simulink model "finalmodel3"  (R2024b)
settings: Solver=ode4  StartTime=0.0  StopTime=110.0  FixedStep=SampleTime  MaxStep=1e-3  RelTol=1e-4  AbsTol=1e-3
PreLoadFcn:
  | load('finalmodel3.mat');
InitFcn:
  | if exist('finalmodel3.mat','file'), load('finalmodel3.mat'); end
values from neighbouring files (symbols this model uses):
  den_d = [1 -0.993736492083]    [finalmodel2.mat]    (also in finalmodel3.mat)
  Dp = 6191.85011148    [finalmodel2.mat]    (also in finalmodel3.mat)
  Dq = 673609.679265    [finalmodel2.mat]    (also in finalmodel3.mat)
  fg = 60    [finalmodel2.mat]    (also in finalmodel3.mat)
  k10 = 1    [finalmodel2.mat]    (also in finalmodel3.mat)
  k11 = 25    [finalmodel2.mat]    (also in finalmodel3.mat)
  k12 = 1    [finalmodel2.mat]    (also in finalmodel3.mat)
  k13 = 120    [finalmodel2.mat]    (also in finalmodel3.mat)
  k14 = 1    [finalmodel2.mat]    (also in finalmodel3.mat)
  k2 = 9.4    [finalmodel2.mat]    (also in finalmodel3.mat)
  k3 = 1    [finalmodel2.mat]    (also in finalmodel3.mat)
  k4 = 25    [finalmodel2.mat]    (also in finalmodel3.mat)
  k5 = 1    [finalmodel2.mat]    (also in finalmodel3.mat)
  k6 = 120    [finalmodel2.mat]    (also in finalmodel3.mat)
  k7 = 1    [finalmodel2.mat]    (also in finalmodel3.mat)
  k9 = 9.4    [finalmodel2.mat]    (also in finalmodel3.mat)
  Ki = 9    [finalmodel2.mat]    (also in finalmodel3.mat)
  Kp = 1    [finalmodel2.mat]    (also in finalmodel3.mat)
  L = 5.78745247607e-06    [finalmodel2.mat]    (also in finalmodel3.mat)
  num_d = [0.00313175395836 0.00313175395836]    [finalmodel2.mat]    (also in finalmodel3.mat)
  Pset = 8281000    [finalmodel2.mat]    (also in finalmodel3.mat = 8280000)
  Qset = 0    [finalmodel2.mat]    (also in finalmodel3.mat)
  R = 0.000290909090909    [finalmodel2.mat]    (also in finalmodel3.mat)
  SampleTime = 5e-05    [finalmodel2.mat]    (also in finalmodel3.mat)
  Ts = 5e-05    [finalmodel2.mat]    (also in finalmodel3.mat)
  tv = 0.05    [finalmodel2.mat]    (also in finalmodel3.mat)
  Vdclink = 800    [finalmodel2.mat]    (also in finalmodel3.mat)
  Vnpeak = 326.598632371    [finalmodel2.mat]    (also in finalmodel3.mat)
  Wn = 376.991118431    [finalmodel2.mat]    (also in finalmodel3.mat)
undefined symbols (not defined in the file or in its folder): dspblkCoreblockFVToolHelper, gcbh, sigbuilder_block
libraries: spsThreePhaseVIMeasurementLib x15, spsLoadFlowBusLib x9, spsThreePhasePISectionLineLib x6, simulink_extras x5, spsThreePhaseTransformerTwoWindingsLib x4, spsThreePhaseParallelRLCLoadLib x4, spsThreePhaseSeriesRLCBranchLib x3, spsSynchronousMachinepuStandardLib x2, spsExcitationSystemLib x2, spsMultiBandPowerSystemStabilizerLib x2, spsSteamTurbineandGovernorLib x2, spsGroundLib x2
(part 2 of 3)

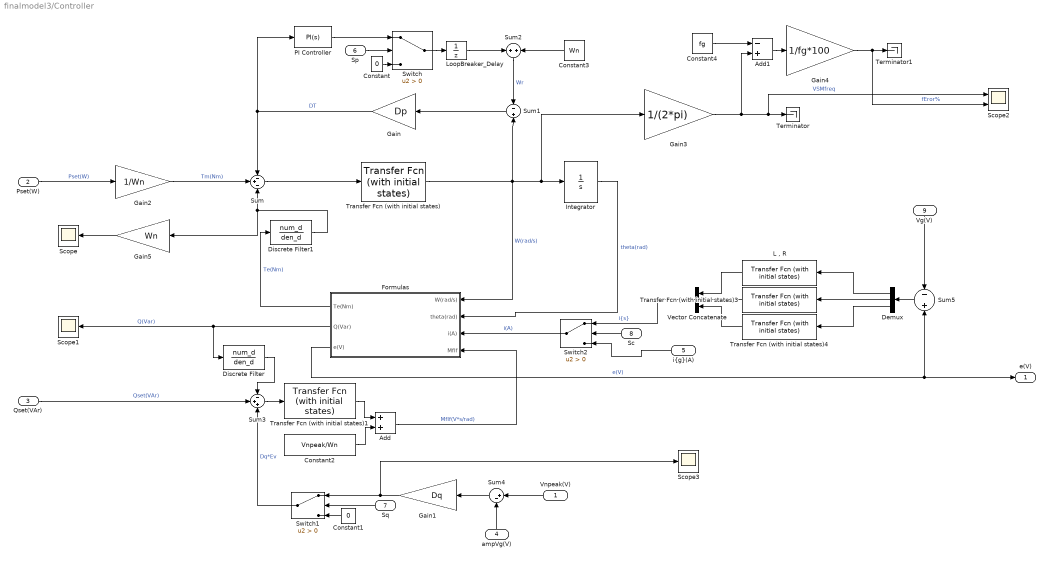
== system finalmodel3/Controller ==
  Vnpeak(V) : Inport  Unit=V
  Pset(W) : Inport  Port=2  Unit=W
  Qset(VAr) : Inport  Port=3  Unit=W
  ampVg(V) : Inport  Port=4  Unit=V
  "i{g}(A)" : Inport  Port=5  Unit=A
  Sp : Inport  Port=6
  Sq : Inport  Port=7
  Sc : Inport  Port=8
  Vg(V) : Inport  Port=9  Unit=V
  Add : Sum
  Add1 : Sum  Inputs=-+
  Constant : Constant  Value=0
  Constant1 : Constant  Value=0
  Constant2 : Constant  Value=Vnpeak/Wn
  Constant3 : Constant  Value=Wn
  Constant4 : Constant  Value=fg
  Demux : Demux  Outputs=3
  Discrete Filter : DiscreteFilter  LoadFcn=dspblkCoreblockFVToolHelper(gcbh,'load');  Numerator=num_d  Denominator=den_d
      settings: CopyFcn=dspblkCoreblockFVToolHelper(gcbh,'copy');  DeleteFcn=dspblkCoreblockFVToolHelper(gcbh,'close');  ModelCloseFcn=dspblkCoreblockFVToolHelper(gcbh,'close');  PreSaveFcn=dspblkCoreblockFVToolHelper(gcbh,'presave');  PostSaveFcn=dspblkCoreblockFVToolHelper(gcbh,'postsave');  CloseFcn=dspblkCoreblockFVToolHelper(gcbh,'close');
  Discrete Filter1 : DiscreteFilter  LoadFcn=dspblkCoreblockFVToolHelper(gcbh,'load');  Numerator=num_d  Denominator=den_d
      settings: CopyFcn=dspblkCoreblockFVToolHelper(gcbh,'copy');  DeleteFcn=dspblkCoreblockFVToolHelper(gcbh,'close');  ModelCloseFcn=dspblkCoreblockFVToolHelper(gcbh,'close');  PreSaveFcn=dspblkCoreblockFVToolHelper(gcbh,'presave');  PostSaveFcn=dspblkCoreblockFVToolHelper(gcbh,'postsave');  CloseFcn=dspblkCoreblockFVToolHelper(gcbh,'close');
  Formulas : Subsystem
  Gain : Gain  Gain=Dp
  Gain1 : Gain  Gain=Dq
  Gain2 : Gain  Gain=1/Wn
  Gain3 : Gain  Gain=1/(2*pi)
  Gain4 : Gain  Gain=1/fg*100
  Gain5 : Gain  Gain=Wn
  Integrator : Integrator  WrapState=on  WrappedStateUpperValue=2*pi  WrappedStateLowerValue=0  ZeroCross=off
  "L , R" : simulink_extras/Additional Linear/Transfer Fcn (with initial states)  N=[1]  D=[L R]  X0=0
  LoopBreaker_Delay : UnitDelay  SampleTime=Ts  HasFrameUpgradeWarning=on
  PI Controller : slpidlib/PID Controller  Controller=PI  Form=Parallel  TimeDomain=Continuous-time  UseExternalTs=off  SampleTime=-1  IntegratorMethod=Forward Euler  FilterMethod=Forward Euler  ControllerParametersSource=internal  P=Kp  I=Ki  UseKiTs=off  D=0  UseExternalDerivativeSource=off  N=100  UseFilter=on  TunerSelectOption=Transfer Function Based (PID Tuner App)  ZeroCross=off  InitialConditionSource=internal  InitialConditionForIntegrator=0  InitialConditionForFilter=0  DifferentiatorICPrevScaledInput=0  ExternalReset=none  TrackingMode=off  Kt=1  LimitOutput=off  SatLimitsSource=internal  UpperSaturationLimit=inf  LowerSaturationLimit=-inf  LinearizeAsGain=on  AntiWindupMode=none  Kb=1  LimitIntegrator=off  UpperIntegratorSaturationLimit=inf  LowerIntegratorSaturationLimit=-inf  POutMin=[]  POutMax=[]  IOutMin=[]  IOutMax=[]  DOutMin=[]  DOutMax=[]  NOutMin=[]  NOutMax=[]  SumOutMin=[]  SumOutMax=[]  SaturationOutMin=[]  SaturationOutMax=[]  PParamMin=[]  PParamMax=[]  IParamMin=[]  IParamMax=[]  DParamMin=[]  DParamMax=[]  NParamMin=[]  NParamMax=[]  KbParamMin=[]  KbParamMax=[]  KtParamMin=[]  KtParamMax=[]  KbOutMin=[]  KbOutMax=[]  KtOutMin=[]  KtOutMax=[]  IntegratorOutMin=[]  IntegratorOutMax=[]  FilterOutMin=[]  FilterOutMax=[]  SumI1OutMin=[]  SumI1OutMax=[]  SumI2OutMin=[]  SumI2OutMax=[]  SumI3OutMin=[]  SumI3OutMax=[]  SumI4OutMin=[]  SumI4OutMax=[]  SumDOutMin=[]  SumDOutMax=[]  DifferentiatorOutMin=[]  DifferentiatorOutMax=[]  FilterDiffOutCoefMin=[]  FilterDiffOutCoefMax=[]  ReciprocalOutMin=[]  ReciprocalOutMax=[]  SumDenOutMin=[]  SumDenOutMax=[]  SumNumOutMin=[]  SumNumOutMax=[]  DivideOutMin=[]  DivideOutMax=[]  UdiffTsProdOutMin=[]  UdiffTsProdOutMax=[]  NTsProdOutMin=[]  NTsProdOutMax=[]  UintegralTsProdOutMin=[]  UintegralTsProdOutMax=[]  UngainTsProdOutMin=[]  UngainTsProdOutMax=[]  ClampingZeroOutDataTypeStr=Inherit: Inherit via back propagation  ClampingZeroOutMin=[]  ClampingZeroOutMax=[]  FilterDenConstantOutDataTypeStr=Inherit: Inherit via back propagation  FilterDenConstantOutMin=[]  FilterDenConstantOutMax=[]  PCopyOutDataTypeStr=Inherit: Inherit via back propagation  PCopyOutMin=[]  PCopyOutMax=[]  NCopyOutDataTypeStr=Inherit: Inherit via back propagation  NCopyOutMin=[]  NCopyOutMax=[]  IntegratorContinuousStateAttributes=''  IntegratorStateMustResolveToSignalObject=off  IntegratorRTWStateStorageClass=Auto  FilterContinuousStateAttributes=''  FilterStateMustResolveToSignalObject=off  FilterRTWStateStorageClass=Auto  ParallelPVariant=InternalParameters  IdealPVariant=Disabled  IVariant=InternalParameters  DVariant=Disabled  IntegratorVariant=Continuous  SatVariant=Disabled  AWVariant=Passthrough  PCopyVariant=Disabled  TRVariant=Disabled  FdbkBlocksVariant=Forward  IdealPFdbkVariant=Disabled  SatFdbkVariant=Disabled  DerivativeFilterVariant=Disabled  NVariant=Disabled  NCopyVariant=Disabled_SignalSpec  FilterICVariant=Disabled  IntegratorICVariant=InternalICs  ExternalResetVariant=Disabled  TRSumVariant=Passthrough  SumFdbkVariant=Disabled  SumVariant=Sum_PI  TsampFilterVariant=InternalTs  TsampNgainVariant=Passthrough  TsampIntegralVariant=Disabled_SignalSpec  ExternalSaturationOutDataTypeStr=Inherit: Same as second input  DerivativeSourceVariant=Disabled  PreIntVariant=InternalPreInt
  Scope : Scope
  Scope1 : Scope
  Scope2 : Scope  NumInputPorts=2
  Scope3 : Scope
  Sum : Sum  Inputs=-+-
  Sum1 : Sum  Inputs=-+
  Sum2 : Sum  Inputs=+|+
  Sum3 : Sum  Inputs=-++
  Sum4 : Sum  Inputs=|+-
  Sum5 : Sum  Inputs=-+
  Switch : Switch  Criteria=u2 > Threshold  SaturateOnIntegerOverflow=off  InputSameDT=off
  Switch1 : Switch  Criteria=u2 > Threshold  SaturateOnIntegerOverflow=off  InputSameDT=off
  Switch2 : Switch  Criteria=u2 > Threshold  SaturateOnIntegerOverflow=off  InputSameDT=off
  Terminator : Terminator
  Terminator1 : Terminator
  Transfer Fcn (with initial states) : simulink_extras/Additional Linear/Transfer Fcn (with initial states)  N=[1]  D=[(tf*Dp) 0]  X0=0
  Transfer Fcn (with initial states)1 : simulink_extras/Additional Linear/Transfer Fcn (with initial states)  N=[1]  D=[tv*Wn*Dq 0]  X0=0
  Transfer Fcn (with initial states)3 : simulink_extras/Additional Linear/Transfer Fcn (with initial states)  N=[1]  D=[L R]  X0=0
  Transfer Fcn (with initial states)4 : simulink_extras/Additional Linear/Transfer Fcn (with initial states)  N=[1]  D=[L R]  X0=0
  Vector Concatenate : Concatenate  NumInputs=3
  e(V) : Outport  Unit=V  VectorParamsAs1DForOutWhenUnconnected=off
  wires:
  Pset(W)/1 -> Gain2/1  "Pset(W)"
  Gain2/1 -> Sum/2  "Tm(Nm)"
  Gain/1 -> PI Controller/1, Sum/1  "DT"
  Sum1/1 -> Gain/1
  PI Controller/1 -> Switch/1
  Sp/1 -> Switch/2
  Constant/1 -> Switch/3
  Sum2/1 -> Sum1/1  "Wr"
  Sum/1 -> Transfer Fcn (with initial states)/1
  Transfer Fcn (with initial states)/1 -> Integrator/1, Gain3/1, Sum1/2, Formulas/1(W(rad/s))  "W(rad/s)"
  Qset(VAr)/1 -> Sum3/2  "Qset(VAr)"
  Formulas/2(Q(Var)) -> Discrete Filter/1, Scope1/1  "Q(Var)"
  Sum3/1 -> Transfer Fcn (with initial states)1/1
  Transfer Fcn (with initial states)1/1 -> Add/1
  Sq/1 -> Switch1/2
  Constant1/1 -> Switch1/3
  Switch1/1 -> Sum3/3  "Dq*Ev"
  Gain1/1 -> Scope3/1, Switch1/1
  Sum4/1 -> Gain1/1
  ampVg(V)/1 -> Sum4/2
  Vnpeak(V)/1 -> Sum4/1
  Sc/1 -> Switch2/2
  "i{g}(A)"/1 -> Switch2/3
  Switch2/1 -> Formulas/3(i(A))  "i(A)"
  Integrator/1 -> Formulas/2(theta(rad))  "theta(rad)"
  Constant3/1 -> Sum2/2
  Vg(V)/1 -> Sum5/1
  Formulas/3(e(V)) -> Sum5/2, e(V)/1  "e(V)"
  Gain3/1 -> Add1/2, Scope2/1, Terminator/1  "VSMfreq"
  Add/1 -> Formulas/4(MfIf)  "MfIf(V*s/rad)"
  Sum5/1 -> Demux/1
  Demux/1 -> "L , R"/1
  Demux/2 -> Transfer Fcn (with initial states)3/1
  Demux/3 -> Transfer Fcn (with initial states)4/1
  Transfer Fcn (with initial states)3/1 -> Vector Concatenate/2
  Vector Concatenate/1 -> Switch2/1  "i{s}"
  "L , R"/1 -> Vector Concatenate/1
  Transfer Fcn (with initial states)4/1 -> Vector Concatenate/3
  Gain4/1 -> Scope2/2, Terminator1/1  "fEror%"
  Add1/1 -> Gain4/1
  Constant4/1 -> Add1/1
  Constant2/1 -> Add/2
  Gain5/1 -> Scope/1
  Discrete Filter/1 -> Sum3/1
  Formulas/1(Te(Nm)) -> Discrete Filter1/1  "Te(Nm)"
  Discrete Filter1/1 -> Gain5/1, Sum/3
  Switch/1 -> LoopBreaker_Delay/1
  LoopBreaker_Delay/1 -> Sum2/1

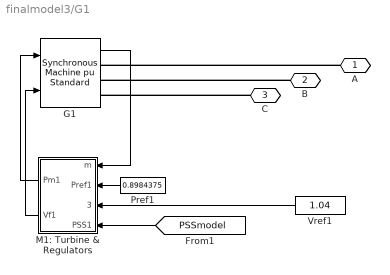
== system finalmodel3/G1 ==
  G1 : spsSynchronousMachinepuStandardLib/Synchronous Machine pu Standard  PresetModel=No  MechanicalLoad=Mechanical power Pm  ShowDetailedParameters=on  RotorType=Round  Units=per unit standard parameters  MeasurementBus=off  NominalParameters="[247.5e6  16500   60 ]"  Reactances1=[1.146 0.2998 0.25 0.969 0.45 0.25 0.025]  Reactances2=[ 1.305, 0.296, 0.252, 0.474, 0.243, 0.18 ]  dAxisTimeConstants=Open-circuit  qAxisTimeConstants=Open-circuit  TimeConstants1=[]  TimeConstants2=[8.96 0.05 0.31 0.05]  TimeConstants3=[]  TimeConstants4=[]  TimeConstants5=[ 1.01, 0.053, 0.1 ]  TimeConstants6=[]  TimeConstants7=[]  TimeConstants8=[]  StatorResistance=0.0025  Mechanical="[ 23.64  0  4]"  PolePairs=4  InitialConditions=[0 -52.9545 0.924925 0.924925 0.924925 -8.45401 -128.454 111.546 1.58772]  SetSaturation=off  Saturation=[0.6404,0.7127,0.8441,0.9214,0.9956,1.082,1.19,1.316,1.457;0.7,0.7698,0.8872,0.9466,0.9969,1.046,1.1,1.151,1.201]  LoadFlowParameters=[2 128000000 0 0 0]  TsPowergui=0  TsBlock=-1  IterativeModel=Trapezoidal non iterative  IterativeDiscreteModel=Trapezoidal non iterative  BusType=swing  Pref=NaN  Qref=0  Qmin=-Inf  Qmax=Inf  PLF=0  QLF=0
      link override Electrical model/Synchronous Machine Discrete Model/Saturation/Lmd_sat/Lmd_sat: SampleTime=SampleTime
      link override Electrical model/Synchronous Machine Discrete Model/Saturation/Lmq_sat/Lmq_sat: SampleTime=SampleTime
      link override Electrical model/Synchronous Machine Discrete Model/phi/Digital Clock: SampleTime=SampleTime
      link override Electrical model/Synchronous Machine Discrete Model/phi/fluxes: SampleTime=SampleTime
      link override Electrical model/Synchronous Machine Discrete Model/phi/voltages: SampleTime=SampleTime
      link override Mechanical model/Delay Prediction/dw_delay: SampleTime=SampleTime
      link override Mechanical model/Delay Prediction/dw_predict: SampleTime=SampleTime
      link override Mechanical model/Digital Clock: SampleTime=SampleTime
      link override Mechanical model/Fcn: Expr=rem(u,2*pi)
      link override Mechanical model/Rotor angle dthetae: SampleTime=SampleTime
      link override Mechanical model/Rotor speed deviation (dw): SampleTime=SampleTime
      link override Mechanical model/theta: SampleTime=SampleTime
  M1: Turbine & Regulators : Subsystem
  Pref1 : Constant  Value=0.8984375  SampleTime=SampleTime
  Vref1 : Constant  Value=1.04  SampleTime=SampleTime
  A : PMIOPort  Side=Left  SampleTime=SampleTime
  B : PMIOPort  Port=2  Side=Left  SampleTime=SampleTime
  C : PMIOPort  Port=3  Side=Left  SampleTime=SampleTime
  wires:
  Pref1/1 -> M1: Turbine & Regulators/2(Pref1)
  [PSSmodel] -> M1: Turbine & Regulators/4(PSS1)
  M1: Turbine & Regulators/1(Pm1) -> G1/1
  M1: Turbine & Regulators/2(Vf1) -> G1/2
  G1/1 -> M1: Turbine & Regulators/1(m)
  Vref1/1 -> M1: Turbine & Regulators/3(Vref1)
  connections:
  A/RConn1 -- G1/RConn1
  B/RConn1 -- G1/RConn2
  C/RConn1 -- G1/RConn3

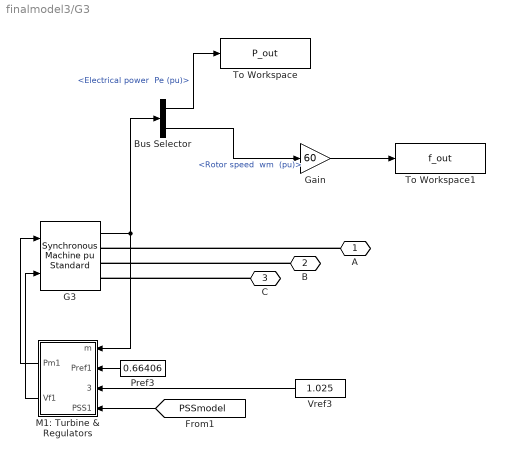
== system finalmodel3/G3 ==
  Bus Selector : BusSelector  OutputSignals="Mechanical.Electrical power  Pe (pu),Mechanical.Rotor speed  wm  (pu)"
  G3 : spsSynchronousMachinepuStandardLib/Synchronous Machine pu Standard  PresetModel=No  MechanicalLoad=Mechanical power Pm  ShowDetailedParameters=on  RotorType=Round  Units=per unit standard parameters  MeasurementBus=off  NominalParameters="[128e6  13800   60 ]"  Reactances1=[1.3125 0.2998 0.25 1.2578 0.45 0.25 0.025]  Reactances2=[ 1.305, 0.296, 0.252, 0.474, 0.243, 0.18 ]  dAxisTimeConstants=Open-circuit  qAxisTimeConstants=Open-circuit  TimeConstants1=[]  TimeConstants2=[5.89 0.05 0.6 0.05]  TimeConstants3=[]  TimeConstants4=[]  TimeConstants5=[ 1.01, 0.053, 0.1 ]  TimeConstants6=[]  TimeConstants7=[]  TimeConstants8=[]  StatorResistance=0.0025  Mechanical="[ 3.01  0  4]"  PolePairs=4  InitialConditions=[0 -58.3097 0.651492 0.651492 0.651492 -3.18103 -123.181 116.819 1.26474]  SetSaturation=off  Saturation=[0.6404,0.7127,0.8441,0.9214,0.9956,1.082,1.19,1.316,1.457;0.7,0.7698,0.8872,0.9466,0.9969,1.046,1.1,1.151,1.201]  LoadFlowParameters=[1 85000000 0 0 0]  TsPowergui=0  TsBlock=-1  IterativeModel=Trapezoidal non iterative  IterativeDiscreteModel=Trapezoidal non iterative  BusType=PV  Pref=85e6  Qref=0  Qmin=-Inf  Qmax=Inf  PLF=0  QLF=0
      link override Electrical model/Synchronous Machine Discrete Model/Saturation/Lmd_sat/Lmd_sat: SampleTime=SampleTime
      link override Electrical model/Synchronous Machine Discrete Model/Saturation/Lmq_sat/Lmq_sat: SampleTime=SampleTime
      link override Electrical model/Synchronous Machine Discrete Model/phi/Digital Clock: SampleTime=SampleTime
      link override Electrical model/Synchronous Machine Discrete Model/phi/fluxes: SampleTime=SampleTime
      link override Electrical model/Synchronous Machine Discrete Model/phi/voltages: SampleTime=SampleTime
      link override Mechanical model/Delay Prediction/dw_delay: SampleTime=SampleTime
      link override Mechanical model/Delay Prediction/dw_predict: SampleTime=SampleTime
      link override Mechanical model/Digital Clock: SampleTime=SampleTime
      link override Mechanical model/Fcn: Expr=rem(u,2*pi)
      link override Mechanical model/Rotor angle dthetae: SampleTime=SampleTime
      link override Mechanical model/Rotor speed deviation (dw): SampleTime=SampleTime
      link override Mechanical model/theta: SampleTime=SampleTime
  Gain : Gain  Gain=60  SampleTime=SampleTime
  M1: Turbine & Regulators : Subsystem
  Pref3 : Constant  Value=0.66406  SampleTime=SampleTime
  To Workspace : ToWorkspace  VariableName=P_out  SaveFormat=Timeseries  SampleTime=SampleTime
  To Workspace1 : ToWorkspace  VariableName=f_out  SaveFormat=Timeseries  SampleTime=SampleTime
  Vref3 : Constant  Value=1.025  SampleTime=SampleTime
  A : PMIOPort  Side=Left  SampleTime=SampleTime
  B : PMIOPort  Port=2  Side=Left  SampleTime=SampleTime
  C : PMIOPort  Port=3  Side=Left  SampleTime=SampleTime
  wires:
  Vref3/1 -> M1: Turbine & Regulators/3(Vref1)
  G3/1 -> Bus Selector/1, M1: Turbine & Regulators/1(m)
  M1: Turbine & Regulators/2(Vf1) -> G3/2
  M1: Turbine & Regulators/1(Pm1) -> G3/1
  [PSSmodel] -> M1: Turbine & Regulators/4(PSS1)
  Pref3/1 -> M1: Turbine & Regulators/2(Pref1)
  Gain/1 -> To Workspace1/1
  Bus Selector/1 -> To Workspace/1  "<Electrical power  Pe (pu)>"
  Bus Selector/2 -> Gain/1  "<Rotor speed  wm  (pu)>"
  connections:
  C/RConn1 -- G3/RConn3
  B/RConn1 -- G3/RConn2
  A/RConn1 -- G3/RConn1

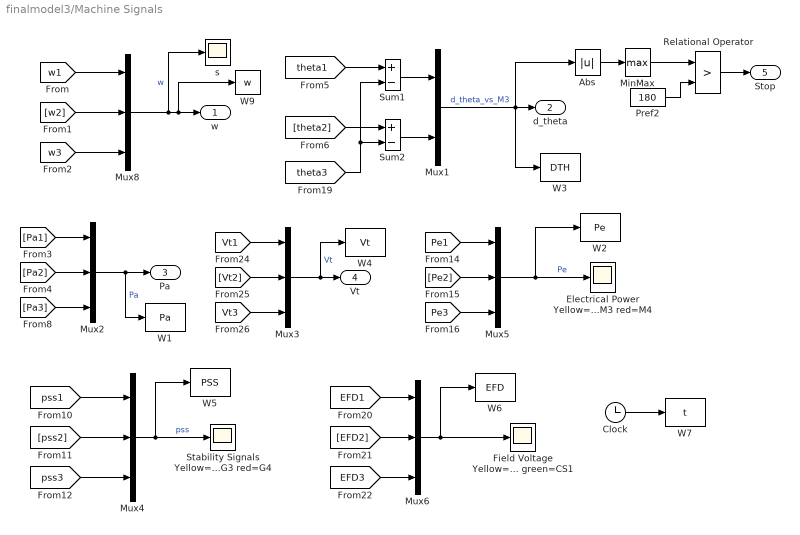
== system finalmodel3/Machine Signals ==
  Abs : Abs  SampleTime=SampleTime
  Clock : Clock
  "Electrical Power Yellow=M1 mag=M2 cyan=M3 red=M4 " : Scope
  Field Voltage Yellow=G1 mag=G2 cyan=G3 red=G4 green=CS1 : Scope
  MinMax : MinMax  Function=max  InputSameDT=on  SaturateOnIntegerOverflow=on  SampleTime=SampleTime
  Mux1 : Mux  Inputs=2
  Mux{2..6,8} (6 alike) : Mux  Inputs=3
  Pref2 : Constant  Value=180  SampleTime=SampleTime
  Relational Operator : RelationalOperator  Operator=>  SampleTime=SampleTime
  "Stability Signals Yellow=G1 mag=G2 cyan=G3 red=G4 " : Scope
  Sum1 : Sum  Inputs=+-  InputSameDT=on  SaturateOnIntegerOverflow=on  SampleTime=SampleTime  OutDataTypeStr=Inherit: Same as first input
  Sum2 : Sum  Inputs=+-  InputSameDT=on  SaturateOnIntegerOverflow=on  SampleTime=SampleTime  OutDataTypeStr=Inherit: Same as first input
  W1 : ToWorkspace  VariableName=Pa  SaveFormat=Timeseries  SampleTime=SampleTime
  W2 : ToWorkspace  VariableName=Pe  SaveFormat=Timeseries  SampleTime=SampleTime
  W3 : ToWorkspace  VariableName=DTH  SaveFormat=Timeseries  SampleTime=SampleTime
  W4 : ToWorkspace  VariableName=Vt  SaveFormat=Timeseries  SampleTime=SampleTime
  W5 : ToWorkspace  VariableName=PSS  SaveFormat=Timeseries  SampleTime=SampleTime
  W6 : ToWorkspace  VariableName=EFD  SaveFormat=Timeseries  SampleTime=SampleTime
  W7 : ToWorkspace  VariableName=t  SaveFormat=Timeseries  SampleTime=SampleTime
  W9 : ToWorkspace  VariableName=w  SaveFormat=Timeseries  SampleTime=SampleTime
  s : Scope
  w : Outport  SampleTime=SampleTime
  d_theta : Outport  Port=2  SampleTime=SampleTime
  Pa : Outport  Port=3  SampleTime=SampleTime
  Vt : Outport  Port=4  SampleTime=SampleTime
  Stop : Outport  Port=5  SampleTime=SampleTime
  wires:
  Mux8/1 -> s/1, W9/1, w/1  "w"
  [w1] -> Mux8/1
  [w2] -> Mux8/2
  [w3] -> Mux8/3
  Mux1/1 -> d_theta/1, Abs/1, W3/1  "d_theta_vs_M3"
  Abs/1 -> MinMax/1
  Pref2/1 -> Relational Operator/2
  MinMax/1 -> Relational Operator/1
  [Pa1] -> Mux2/1
  Mux4/1 -> "Stability Signals Yellow=G1 mag=G2 cyan=G3 red=G4 "/1, W5/1  "pss"
  [pss1] -> Mux4/1
  [pss2] -> Mux4/2
  [pss3] -> Mux4/3
  [EFD1] -> Mux6/1
  [EFD2] -> Mux6/2
  [EFD3] -> Mux6/3
  Mux6/1 -> Field Voltage Yellow=G1 mag=G2 cyan=G3 red=G4 green=CS1/1, W6/1
  Relational Operator/1 -> Stop/1
  Mux2/1 -> Pa/1, W1/1  "Pa"
  [theta1] -> Sum1/1
  Sum1/1 -> Mux1/1
  [theta2] -> Sum2/1
  [theta3] -> Sum1/2, Sum2/2
  Sum2/1 -> Mux1/2
  [Pa2] -> Mux2/2
  [Pa3] -> Mux2/3
  [Vt1] -> Mux3/1
  [Vt2] -> Mux3/2
  [Vt3] -> Mux3/3
  Mux3/1 -> Vt/1, W4/1  "Vt"
  [Pe1] -> Mux5/1
  [Pe2] -> Mux5/2
  [Pe3] -> Mux5/3
  Mux5/1 -> "Electrical Power Yellow=M1 mag=M2 cyan=M3 red=M4 "/1, W2/1  "Pe"
  Clock/1 -> W7/1

== system finalmodel3/Signal Builder2 ==
  Demux : Demux  Tag=STV Demux  Outputs=1
      settings: DisplayOption=none
  FromWs : FromWorkspace  Tag=STV FromWs  VariableName=tuvar
      SigBuilderData=|
      | common.afterFinalStr = 'Extrapolate'
      | common.sampleTime = 0
      | dataSet.timeRange = [0 4]
      | dataSet.name = 'Group 1'
      | sbobj.Groups.Name = 'Group 1'
      | sbobj.Groups.Signals.Name = 'Signal 1'
      | sbobj.Groups.Signals.XData = [0 0.00416233090531 0.00832466181061 0.0124869927159 0.0166493236212 0.0208116545265 0.0249739854318 0.0291363163371 0.0332986472425 0.0374609781478 0.0416233090531 0.0457856399584 ... (962 elements, 1x962)]
      | sbobj.Groups.Signals.YData = [2.47122187864 2.47122187864 2.47122187864 2.47122187864 2.47122187864 2.47122187864 2.47122187864 2.47122187864 2.47122187864 2.47121149505 2.47121149505 2.47121149505 ... (962 elements, 1x962)]
      | sbobj.Groups.TimeRange = [0 4]
  Signal 1 : Outport  Tag=STV Outport  VectorParamsAs1DForOutWhenUnconnected=off
  wires:
  FromWs/1 -> Demux/1
  Demux/1 -> Signal 1/1

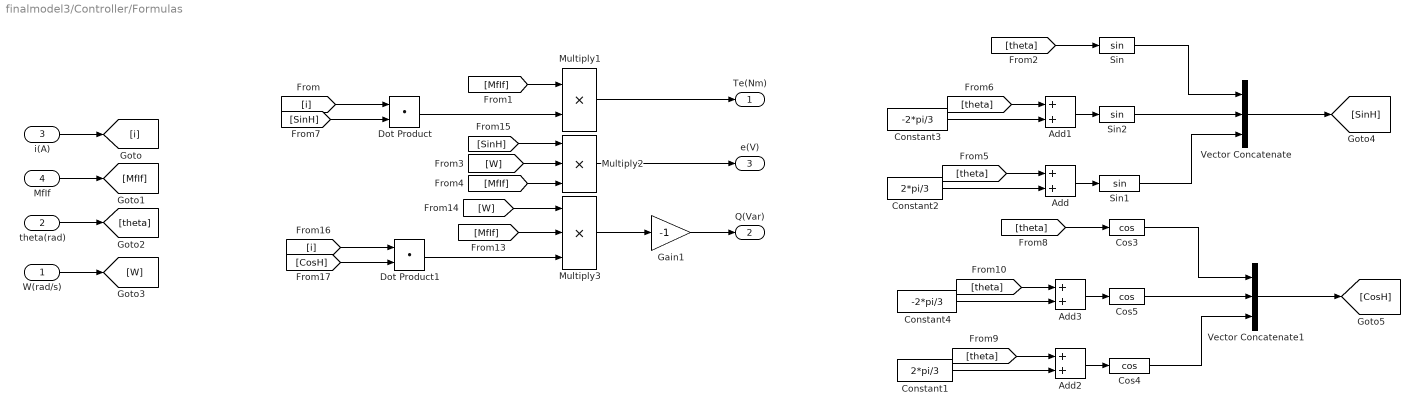
== system finalmodel3/Controller/Formulas ==
  W(rad/s) : Inport  Unit=rad/s
  theta(rad) : Inport  Port=2  Unit=rad
  i(A) : Inport  Port=3  Unit=A
  MfIf : Inport  Port=4  Unit=V*s/rad
  Add{,1..3} (4 alike) : Sum
  Constant1 : Constant  Value=2*pi/3
  Constant2 : Constant  Value=2*pi/3
  Constant3 : Constant  Value=-2*pi/3
  Constant4 : Constant  Value=-2*pi/3
  Cos3 : Trigonometry  Operator=cos
  Cos4 : Trigonometry  Operator=cos
  Cos5 : Trigonometry  Operator=cos
  Dot Product : DotProduct  OutDataTypeStr=Inherit: Inherit via internal rule
  Dot Product1 : DotProduct  OutDataTypeStr=Inherit: Inherit via internal rule
  Gain1 : Gain  Gain=-1
  Multiply1 : Product
  Multiply2 : Product  Inputs=3
  Multiply3 : Product  Inputs=3
  Sin : Trigonometry
  Sin1 : Trigonometry
  Sin2 : Trigonometry
  Vector Concatenate : Concatenate  NumInputs=3
  Vector Concatenate1 : Concatenate  NumInputs=3
  Te(Nm) : Outport  Unit=N*m  VectorParamsAs1DForOutWhenUnconnected=off
  Q(Var) : Outport  Port=2  Unit=W  VectorParamsAs1DForOutWhenUnconnected=off
  e(V) : Outport  Port=3  Unit=V  VectorParamsAs1DForOutWhenUnconnected=off
  wires:
  Multiply3/1 -> Gain1/1
  Multiply1/1 -> Te(Nm)/1
  Constant2/1 -> Add/2
  Constant3/1 -> Add1/2
  Gain1/1 -> Q(Var)/1
  i(A)/1 -> [i]
  MfIf/1 -> [MfIf]
  theta(rad)/1 -> [theta]
  W(rad/s)/1 -> [W]
  [theta] -> Sin/1
  [MfIf] -> Multiply1/1
  [W] -> Multiply2/2
  [MfIf] -> Multiply2/3
  Multiply2/1 -> e(V)/1
  [theta] -> Add/1
  [theta] -> Add1/1
  Add/1 -> Sin1/1
  Add1/1 -> Sin2/1
  [MfIf] -> Multiply3/2
  Sin2/1 -> Vector Concatenate/2
  Sin/1 -> Vector Concatenate/1
  Sin1/1 -> Vector Concatenate/3
  Vector Concatenate/1 -> [SinH]
  [SinH] -> Multiply2/1
  [i] -> Dot Product/1
  [SinH] -> Dot Product/2
  Dot Product/1 -> Multiply1/2
  Cos5/1 -> Vector Concatenate1/2
  Vector Concatenate1/1 -> [CosH]
  Add2/1 -> Cos4/1
  Constant4/1 -> Add3/2
  Cos4/1 -> Vector Concatenate1/3
  Constant1/1 -> Add2/2
  [theta] -> Add2/1
  Add3/1 -> Cos5/1
  [theta] -> Add3/1
  Cos3/1 -> Vector Concatenate1/1
  [theta] -> Cos3/1
  [i] -> Dot Product1/1
  [CosH] -> Dot Product1/2
  [W] -> Multiply3/1
  Dot Product1/1 -> Multiply3/3

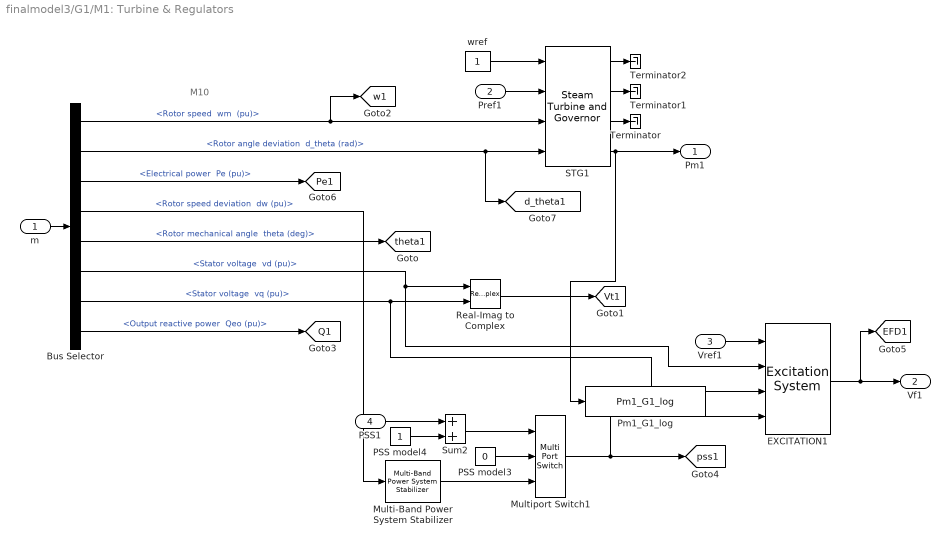
== system finalmodel3/G1/M1: Turbine & Regulators ==
  note: M10
  m : Inport  SampleTime=SampleTime
  Pref1 : Inport  Port=2  SampleTime=SampleTime
  Vref1 : Inport  Port=3  SampleTime=SampleTime
  PSS1 : Inport  Port=4  SampleTime=SampleTime
  Bus Selector : BusSelector  OutputSignals="Mechanical.Rotor speed  wm  (pu),Mechanical.Rotor angle deviation  d_theta (rad),Mechanical.Electrical power  Pe (pu),Mechanical.Rotor speed deviation  dw (pu),Mechanical.Rotor mechanical angle  theta (deg),dq0 components.Stator voltage  vd (pu),dq0 components.Stator voltage  vq (pu),Output reactive power  Qeo (pu)"
  EXCITATION1 : spsExcitationSystemLib/Excitation System  tr=0.01  reg=[20 0.2 ]  exc=[ 1, 0.314 ]  tgr=[10 1]  damp=[ 0, 0 ]  sat=[ 0, 0 ]  lim="[-5 5  0 ]"  v0=[1.04 1.5877]
      link override Model: Ts=SampleTime
      link override Model/Damping kfd.s // (tfd.s +1)/1st-Order Discrete Filter: Ts=SampleTime
      link override Model/Damping kfd.s // (tfd.s +1)/1st-Order Discrete Filter/Discrete State-Space: SampleTime=SampleTime
      link override Model/Exciter  1 // (te.s + ke)/1st order Lowpass: Ts=SampleTime
      link override Model/Exciter  1 // (te.s + ke)/1st order Lowpass/Discrete State-Space: SampleTime=SampleTime
      link override Model/Lead Lag Compensator tc.s+1 // tb.s+1: Ts=SampleTime
      link override Model/Lead Lag Compensator tc.s+1 // tb.s+1/Discrete State-Space: SampleTime=SampleTime
      link override Model/Low Pass Filter 1 // (tr.s +1) (with IC): Ts=SampleTime
      link override Model/Low Pass Filter 1 // (tr.s +1) (with IC)/Discrete State-Space: SampleTime=SampleTime
      link override Model/Main Regulator ka // (ta.s +1)/1st order Lowpass: Ts=SampleTime
      link override Model/Main Regulator ka // (ta.s +1)/1st order Lowpass/Discrete State-Space: SampleTime=SampleTime
      link override Model/Positive Sequence Voltage: Expr=sqrt(abs(u(1)^2 + u(2)^2))
      link override Model/Unit Delay1: SampleTime=SampleTime
      link override Model/Unit Delay2: SampleTime=SampleTime
      settings: LibrarySourceBlock=sps_lib/Electrical Machines/Synchronous Machine Control/Excitation System
  Multi-Band Power System Stabilizer : spsMultiBandPowerSystemStabilizerLib/Multi-Band Power System Stabilizer  OperationMode=Simplified settings  Kg=k8  GL=[k9 k10]  GI=[k11 k12]  GH=[k13 k14]  GLd=[66 66 9.4]  TcLF=[1.667 2 0 0 0 0 2 2.4 0 0 0 0 1 1]  GId=[66 66 47.6]  TcIF=[1 1 0.25 0.3 0 0 1 1 0.3 0.36 0 0 0 0]  GHd=[66 66 233]  TcHF="[0.01 0.012 0 0 0 0  0.012 0.0144 0 0 0 0 1 1]"  LIM=[.075 .15 .15 .15]  Plot_On=off  MagdB_On=off  FreqRange=logspace(-2,2,500)
      link override Model/Discrete Lead-Lag1: Ts=SampleTime
      link override Model/Discrete Lead-Lag1/Discrete State-Space: SampleTime=SampleTime
      link override Model/Discrete Lead-Lag2: Ts=SampleTime
      link override Model/Discrete Lead-Lag2/Discrete State-Space: SampleTime=SampleTime
      link override Model/Discrete Lead-Lag3: Ts=SampleTime
      link override Model/Discrete Lead-Lag3/Discrete State-Space: SampleTime=SampleTime
      link override Model/Discrete Lead-Lag4: Ts=SampleTime
      link override Model/Discrete Lead-Lag4/Discrete State-Space: SampleTime=SampleTime
      link override Model/Discrete Lead-Lag5: Ts=SampleTime
      link override Model/Discrete Lead-Lag5/Discrete State-Space: SampleTime=SampleTime
      link override Model/Discrete Lead-Lag6: Ts=SampleTime
      link override Model/Discrete Lead-Lag6/Discrete State-Space: SampleTime=SampleTime
      link override Model/HF speed sensor: Ts=SampleTime
      link override Model/HF speed sensor/Discrete State-Space: SampleTime=SampleTime
      link override Model/LF and IF speed sensor: Ts=SampleTime
      link override Model/LF and IF speed sensor/Discrete State-Space: SampleTime=SampleTime
      link override Model/Transfer function for detailed model (HF)/Transfer functions for detailed stabilizer/Discrete Lead-Lag1: Ts=SampleTime
      link override Model/Transfer function for detailed model (HF)/Transfer functions for detailed stabilizer/Discrete Lead-Lag1/Discrete State-Space: SampleTime=SampleTime
      link override Model/Transfer function for detailed model (HF)/Transfer functions for detailed stabilizer/Discrete Lead-Lag2: Ts=SampleTime
      link override Model/Transfer function for detailed model (HF)/Transfer functions for detailed stabilizer/Discrete Lead-Lag2/Discrete State-Space: SampleTime=SampleTime
      link override Model/Transfer function for detailed model (HF)/Transfer functions for detailed stabilizer1/Discrete Lead-Lag1: Ts=SampleTime
      link override Model/Transfer function for detailed model (HF)/Transfer functions for detailed stabilizer1/Discrete Lead-Lag1/Discrete State-Space: SampleTime=SampleTime
      link override Model/Transfer function for detailed model (HF)/Transfer functions for detailed stabilizer1/Discrete Lead-Lag2: Ts=SampleTime
      link override Model/Transfer function for detailed model (HF)/Transfer functions for detailed stabilizer1/Discrete Lead-Lag2/Discrete State-Space: SampleTime=SampleTime
      link override Model/Transfer function for detailed model (IF)/Transfer functions for detailed stabilizer/Discrete Lead-Lag1: Ts=SampleTime
      link override Model/Transfer function for detailed model (IF)/Transfer functions for detailed stabilizer/Discrete Lead-Lag1/Discrete State-Space: SampleTime=SampleTime
      link override Model/Transfer function for detailed model (IF)/Transfer functions for detailed stabilizer/Discrete Lead-Lag2: Ts=SampleTime
      link override Model/Transfer function for detailed model (IF)/Transfer functions for detailed stabilizer/Discrete Lead-Lag2/Discrete State-Space: SampleTime=SampleTime
      link override Model/Transfer function for detailed model (IF)/Transfer functions for detailed stabilizer1/Discrete Lead-Lag1: Ts=SampleTime
      link override Model/Transfer function for detailed model (IF)/Transfer functions for detailed stabilizer1/Discrete Lead-Lag1/Discrete State-Space: SampleTime=SampleTime
      link override Model/Transfer function for detailed model (IF)/Transfer functions for detailed stabilizer1/Discrete Lead-Lag2: Ts=SampleTime
      link override Model/Transfer function for detailed model (IF)/Transfer functions for detailed stabilizer1/Discrete Lead-Lag2/Discrete State-Space: SampleTime=SampleTime
      link override Model/Transfer function for detailed model (LF)/Transfer functions for detailed stabilizer/Discrete Lead-Lag1: Ts=SampleTime
      link override Model/Transfer function for detailed model (LF)/Transfer functions for detailed stabilizer/Discrete Lead-Lag1/Discrete State-Space: SampleTime=SampleTime
      link override Model/Transfer function for detailed model (LF)/Transfer functions for detailed stabilizer/Discrete Lead-Lag2: Ts=SampleTime
      link override Model/Transfer function for detailed model (LF)/Transfer functions for detailed stabilizer/Discrete Lead-Lag2/Discrete State-Space: SampleTime=SampleTime
      link override Model/Transfer function for detailed model (LF)/Transfer functions for detailed stabilizer1/Discrete Lead-Lag1: Ts=SampleTime
      link override Model/Transfer function for detailed model (LF)/Transfer functions for detailed stabilizer1/Discrete Lead-Lag1/Discrete State-Space: SampleTime=SampleTime
      link override Model/Transfer function for detailed model (LF)/Transfer functions for detailed stabilizer1/Discrete Lead-Lag2: Ts=SampleTime
      link override Model/Transfer function for detailed model (LF)/Transfer functions for detailed stabilizer1/Discrete Lead-Lag2/Discrete State-Space: SampleTime=SampleTime
      settings: LibrarySourceBlock=|
      | sps_lib/Electrical Machines/Synchronous Machine Control/Multi-Band
      | Power System Stabilizer
  Multiport Switch1 : MultiPortSwitch  Inputs=2  SampleTime=SampleTime  SaturateOnIntegerOverflow=off
  PSS model3 : Constant  Value=0  SampleTime=SampleTime
  PSS model4 : Constant  SampleTime=SampleTime
  Pm1_G1_log : ToWorkspace  VariableName=Pm1_G1_log  SaveFormat=Timeseries  SampleTime=-1
  Real-Imag to Complex : RealImagToComplex  SampleTime=SampleTime
  STG1 : spsSteamTurbineandGovernorLib/Steam Turbine and Governor  gentype=Tandem-compound (single mass)  reg1="[ 1  0.05    0 ]"  reg2="[ 0.001  0.15 ]"  reg3="[ -0.1  0.1  0  4.496 ]"  N=3600  turb1="[ 0  10   3.3   0.5   ]"  turb2="[   0   0.36    0.36   0.28   ]"  HA="[ 0.046  1.430  1.465   0.192 ]"  KA="[ 90.44  53.88  64.59   62.94  ]"  DA="[ 0.0115  0.3575  0.3663   0.0137  ]"  ini1=0.95361  ini2=[0.779316,-31.4247]
      link override Model/4 mass shaft/1 mass/Mass2: Ts=SampleTime
      link override Model/4 mass shaft/1 mass/Mass2/Ad*x(k-1): SampleTime=SampleTime
      link override Model/4 mass shaft/1 mass/Mass2/Bd*(u(k)+ u(k-1)): SampleTime=SampleTime
      link override Model/4 mass shaft/1 mass/Mass2/Delay_u: SampleTime=SampleTime
      link override Model/4 mass shaft/1 mass/Mass2/Delay_x: SampleTime=SampleTime
      link override Model/4 mass shaft/1 mass/Mass2/Digital Clock: SampleTime=SampleTime
      link override Model/4 mass shaft/1 mass/Mass2/Prediction/Unit Delay3: SampleTime=SampleTime
      link override Model/4 mass shaft/2 masses/Mass2: Ts=SampleTime
      link override Model/4 mass shaft/2 masses/Mass2/Ad*x(k-1): SampleTime=SampleTime
      link override Model/4 mass shaft/2 masses/Mass2/Bd*(u(k)+ u(k-1)): SampleTime=SampleTime
      link override Model/4 mass shaft/2 masses/Mass2/Delay_u: SampleTime=SampleTime
      link override Model/4 mass shaft/2 masses/Mass2/Delay_x: SampleTime=SampleTime
      link override Model/4 mass shaft/2 masses/Mass2/Digital Clock: SampleTime=SampleTime
      link override Model/4 mass shaft/2 masses/Mass2/Prediction/Unit Delay3: SampleTime=SampleTime
      link override Model/4 mass shaft/2 masses/Mass3: Ts=SampleTime
      link override Model/4 mass shaft/2 masses/Mass3/Ad*x(k-1): SampleTime=SampleTime
      link override Model/4 mass shaft/2 masses/Mass3/Bd*(u(k)+ u(k-1)): SampleTime=SampleTime
      link override Model/4 mass shaft/2 masses/Mass3/Delay_u: SampleTime=SampleTime
      link override Model/4 mass shaft/2 masses/Mass3/Delay_x: SampleTime=SampleTime
      link override Model/4 mass shaft/2 masses/Mass3/Digital Clock: SampleTime=SampleTime
      link override Model/4 mass shaft/2 masses/Mass3/Prediction/Unit Delay3: SampleTime=SampleTime
      link override Model/4 mass shaft/3 masses/Mass2: Ts=SampleTime
      link override Model/4 mass shaft/3 masses/Mass2/Ad*x(k-1): SampleTime=SampleTime
      link override Model/4 mass shaft/3 masses/Mass2/Bd*(u(k)+ u(k-1)): SampleTime=SampleTime
      link override Model/4 mass shaft/3 masses/Mass2/Delay_u: SampleTime=SampleTime
      link override Model/4 mass shaft/3 masses/Mass2/Delay_x: SampleTime=SampleTime
      link override Model/4 mass shaft/3 masses/Mass2/Digital Clock: SampleTime=SampleTime
      link override Model/4 mass shaft/3 masses/Mass2/Prediction/Unit Delay3: SampleTime=SampleTime
      link override Model/4 mass shaft/3 masses/Mass3: Ts=SampleTime
      link override Model/4 mass shaft/3 masses/Mass3/Ad*x(k-1): SampleTime=SampleTime
      link override Model/4 mass shaft/3 masses/Mass3/Bd*(u(k)+ u(k-1)): SampleTime=SampleTime
      link override Model/4 mass shaft/3 masses/Mass3/Delay_u: SampleTime=SampleTime
      link override Model/4 mass shaft/3 masses/Mass3/Delay_x: SampleTime=SampleTime
      link override Model/4 mass shaft/3 masses/Mass3/Digital Clock: SampleTime=SampleTime
      link override Model/4 mass shaft/3 masses/Mass3/Prediction/Unit Delay3: SampleTime=SampleTime
      link override Model/4 mass shaft/3 masses/Mass4: Ts=SampleTime
      link override Model/4 mass shaft/3 masses/Mass4/Ad*x(k-1): SampleTime=SampleTime
      link override Model/4 mass shaft/3 masses/Mass4/Bd*(u(k)+ u(k-1)): SampleTime=SampleTime
      link override Model/4 mass shaft/3 masses/Mass4/Delay_u: SampleTime=SampleTime
      link override Model/4 mass shaft/3 masses/Mass4/Delay_x: SampleTime=SampleTime
      link override Model/4 mass shaft/3 masses/Mass4/Digital Clock: SampleTime=SampleTime
      link override Model/4 mass shaft/3 masses/Mass4/Prediction/Unit Delay3: SampleTime=SampleTime
      link override Model/4 mass shaft/4 masses/Mass2: Ts=SampleTime
      link override Model/4 mass shaft/4 masses/Mass2/Ad*x(k-1): SampleTime=SampleTime
      link override Model/4 mass shaft/4 masses/Mass2/Bd*(u(k)+ u(k-1)): SampleTime=SampleTime
      link override Model/4 mass shaft/4 masses/Mass2/Delay_u: SampleTime=SampleTime
      link override Model/4 mass shaft/4 masses/Mass2/Delay_x: SampleTime=SampleTime
      link override Model/4 mass shaft/4 masses/Mass2/Digital Clock: SampleTime=SampleTime
      link override Model/4 mass shaft/4 masses/Mass2/Prediction/Unit Delay3: SampleTime=SampleTime
      link override Model/4 mass shaft/4 masses/Mass3: Ts=SampleTime
      link override Model/4 mass shaft/4 masses/Mass3/Ad*x(k-1): SampleTime=SampleTime
      link override Model/4 mass shaft/4 masses/Mass3/Bd*(u(k)+ u(k-1)): SampleTime=SampleTime
      link override Model/4 mass shaft/4 masses/Mass3/Delay_u: SampleTime=SampleTime
      link override Model/4 mass shaft/4 masses/Mass3/Delay_x: SampleTime=SampleTime
      link override Model/4 mass shaft/4 masses/Mass3/Digital Clock: SampleTime=SampleTime
      link override Model/4 mass shaft/4 masses/Mass3/Prediction/Unit Delay3: SampleTime=SampleTime
      link override Model/4 mass shaft/4 masses/Mass4: Ts=SampleTime
      link override Model/4 mass shaft/4 masses/Mass4/Ad*x(k-1): SampleTime=SampleTime
      link override Model/4 mass shaft/4 masses/Mass4/Bd*(u(k)+ u(k-1)): SampleTime=SampleTime
      link override Model/4 mass shaft/4 masses/Mass4/Delay_u: SampleTime=SampleTime
      link override Model/4 mass shaft/4 masses/Mass4/Delay_x: SampleTime=SampleTime
      link override Model/4 mass shaft/4 masses/Mass4/Digital Clock: SampleTime=SampleTime
      link override Model/4 mass shaft/4 masses/Mass4/Prediction/Unit Delay3: SampleTime=SampleTime
      link override Model/4 mass shaft/4 masses/Mass5: Ts=SampleTime
      link override Model/4 mass shaft/4 masses/Mass5/Ad*x(k-1): SampleTime=SampleTime
      link override Model/4 mass shaft/4 masses/Mass5/Bd*(u(k)+ u(k-1)): SampleTime=SampleTime
      link override Model/4 mass shaft/4 masses/Mass5/Delay_u: SampleTime=SampleTime
      link override Model/4 mass shaft/4 masses/Mass5/Delay_x: SampleTime=SampleTime
      link override Model/4 mass shaft/4 masses/Mass5/Digital Clock: SampleTime=SampleTime
      link override Model/4 mass shaft/4 masses/Mass5/Prediction/Unit Delay3: SampleTime=SampleTime
      link override Model/speed regulator/Servo-motor Position: SampleTime=SampleTime
      link override Model/speed regulator/Speed Relay: Ts=SampleTime
      link override Model/speed regulator/Speed Relay/In: SampleTime=SampleTime
      link override Model/speed regulator/Speed Relay/Model/Delay_x: SampleTime=SampleTime
      link override Model/speed regulator/Speed Relay/Out: SampleTime=SampleTime
      link override Model/steam turbine/Stage 1/Constant4: SampleTime=SampleTime
      link override Model/steam turbine/Stage 1/Stage1/Stage1: Ts=SampleTime
      link override Model/steam turbine/Stage 1/Stage1/Stage1/In: SampleTime=SampleTime
      link override Model/steam turbine/Stage 1/Stage1/Stage1/Model/Delay_x: SampleTime=SampleTime
      link override Model/steam turbine/Stage 1/Stage1/Stage1/Out: SampleTime=SampleTime
      link override Model/steam turbine/Stage 2 /Constant3: SampleTime=SampleTime
      link override Model/steam turbine/Stage 2 /Stage2/Stage2: Ts=SampleTime
      link override Model/steam turbine/Stage 2 /Stage2/Stage2/In: SampleTime=SampleTime
      link override Model/steam turbine/Stage 2 /Stage2/Stage2/Model/Delay_x: SampleTime=SampleTime
      link override Model/steam turbine/Stage 2 /Stage2/Stage2/Out: SampleTime=SampleTime
      link override Model/steam turbine/Stage 3/Constant2: SampleTime=SampleTime
      link override Model/steam turbine/Stage 3/Stage3/Stage3: Ts=SampleTime
      link override Model/steam turbine/Stage 3/Stage3/Stage3/In: SampleTime=SampleTime
      link override Model/steam turbine/Stage 3/Stage3/Stage3/Model/Delay_x: SampleTime=SampleTime
      link override Model/steam turbine/Stage 3/Stage3/Stage3/Out: SampleTime=SampleTime
      link override Model/steam turbine/Stage 4/Constant1: SampleTime=SampleTime
      link override Model/steam turbine/Stage 4/Stage4/Stage4: Ts=SampleTime
      link override Model/steam turbine/Stage 4/Stage4/Stage4/In: SampleTime=SampleTime
      link override Model/steam turbine/Stage 4/Stage4/Stage4/Model/Delay_x: SampleTime=SampleTime
      link override Model/steam turbine/Stage 4/Stage4/Stage4/Out: SampleTime=SampleTime
      settings: LibrarySourceBlock=|
      | sps_lib/Electrical Machines/Synchronous Machine Control/Steam Turbine
      | and Governor
  Sum2 : Sum  InputSameDT=on  SaturateOnIntegerOverflow=on  SampleTime=SampleTime  OutDataTypeStr=Inherit: Same as first input
  Terminator : Terminator
  Terminator1 : Terminator
  Terminator2 : Terminator
  wref : Constant  SampleTime=SampleTime
  Pm1 : Outport  SampleTime=SampleTime  InitialOutput=0
  Vf1 : Outport  Port=2  SampleTime=SampleTime  InitialOutput=0
  tag scope: EFD1=global, Pe1=global, Q1=global, Vt1=global, d_theta1=global, pss1=global, theta1=global, w1=global
  wires:
  Bus Selector/7 -> EXCITATION1/3, Real-Imag to Complex/2  "<Stator voltage  vq (pu)>"
  wref/1 -> STG1/1
  Pref1/1 -> STG1/2
  m/1 -> Bus Selector/1
  Vref1/1 -> EXCITATION1/1
  EXCITATION1/1 -> Vf1/1, [EFD1]
  Real-Imag to Complex/1 -> [Vt1]
  Bus Selector/5 -> [theta1]  "<Rotor mechanical angle  theta (deg)>"
  Bus Selector/6 -> Real-Imag to Complex/1, EXCITATION1/2  "<Stator voltage  vd (pu)>"
  STG1/3 -> Terminator/1
  STG1/4 -> Pm1/1, Pm1_G1_log/1
  STG1/2 -> Terminator1/1
  STG1/1 -> Terminator2/1
  Bus Selector/1 -> [w1], STG1/3  "<Rotor speed  wm  (pu)>"
  Bus Selector/2 -> [d_theta1], STG1/4  "<Rotor angle deviation  d_theta (rad)>"
  Bus Selector/3 -> [Pe1]  "<Electrical power  Pe (pu)>"
  Bus Selector/8 -> [Q1]  "<Output reactive power  Qeo (pu)>"
  PSS1/1 -> Sum2/1
  Sum2/1 -> Multiport Switch1/1
  PSS model4/1 -> Sum2/2
  Multi-Band Power System Stabilizer/1 -> Multiport Switch1/3
  PSS model3/1 -> Multiport Switch1/2
  Multiport Switch1/1 -> [pss1], EXCITATION1/4
  Bus Selector/4 -> Multi-Band Power System Stabilizer/1  "<Rotor speed deviation  dw (pu)>"
